simulink model "A_OnTheGo_PID"  (R2026a)
settings: Solver=daessc  StopTime=10
undefined symbols (not defined in the file): motor, RotateMass, X, Y, Z
libraries: sm_lib x823, nesl_utility x31, simulink x1
(part 1 of 25)
settings Model: Creator=fdors  LastModifiedBy=ctalle16
settings SimscapeCC: SimscapeNominalValues="[{\"value\":\"1\",\"unit\":\"A\"},{\"value\":\"1\",\"unit\":\"bar\"},{\"value\":\"1\",\"unit\":\"cm^2\"},{\"value\":\"1\",\"unit\":\"cm^3/s\"},{\"value\":\"1\",\"unit\":\"kJ/kg\"},{\"value\":\"1\",\"unit\":\"kW\"},{\"value\":\"1\",\"unit\":\"l\"},{\"value\":\"1\",\"unit\":\"N\"},{\"value\":\"1\",\"unit\":\"N*m\"},{\"value\":\"1\",\"unit\":\"V\"}]"  SimscapeLogType=none  SimscapeLogDataHistory=5000.0
settings ExplorerConfigSet: InternalSimMechanicsExplorerSettings=|
  | <ExplorerConfiguration>
  | 
  |   <canonicalview>planar_xy</canonicalview>
  | 
  |   <TilePanel>
  |     <TileInfo>
  |       <Tiles Columns="1" Count="1" Height="985" Rows="1" Width="1142">
  |         <Row Weight="1"/>
  |         <Column Weight="1"/>
  |         <Tile Height="1" Width="1" X="0" Y="0"/>
  |       </Tiles>
  |     </TileInfo>
  |     <SceneInfo>
  |       <SceneViewer>
  |         <IsThisViewStd>
  |           <IsStandardView>off</IsStandardView>
  |           <StandardViewName>Front</StandardViewName>
  |         </IsThisViewStd>
  |         <BGColor>
  |           <R>1</R>
  |           <G>1</G>
  |           <B>1</B>
  |           <A>1</A>
  |         </BGColor>
  |         <Camera>
  |           <DoPerspective>off</DoPerspective>
  |           <Position>
  |             <X>0.67806105182753051</X>
  |             <Y>0.74872215079128168</Y>
  |             <Z>0.72031476009846773</Z>
  |           </Position>
  |           <Center>
  |             <X>-0.014616720378398888</X>
  |             <Y>0.056044378585352252</Y>
  |             <Z>0.027636987892538302</Z>
  |           </Center>
  |           <Up>
  |             <X>-0.40824829046386302</X>
  |             <Y>0.81649658092772603</Y>
  |             <Z>-0.40824829046386302</Z>
  |           </Up>
  |           <XLim>0.17072201332507064</XLim>
  |           <YLim>0.17072201332507064</YLim>
  |           <ViewLimDist>0.01</ViewLimDist>
  |         </Camera>
  |       </SceneViewer>
  |     </SceneInfo>
  |   </TilePanel>
  | 
  |   <MechEditorPanel>
  |     <GfxPanelCameraMap/>
  |     <Cameras/>
  |     <VideoCreator>
  |       <IncludeTiles>All</IncludeTiles>
  |       <IncludeTime>on</IncludeTime>
  |       <IncludeWorldFrame>off</IncludeWorldFrame>
  |       <PlaybackSpeedRatio>1</PlaybackSpeedRatio>
  |       <FrameRate>30</FrameRate>
  |       <FrameSize>auto</FrameSize>
  |       <VideoFormat>UncompressedAVI</VideoFormat>
  |     </VideoCreator>
  |   </MechEditorPanel>
  | 
  |   <PlaybackSettings>
  |     <PlaybackSpeedFactor>1</PlaybackSpeedFactor>
  |   </PlaybackSettings>
  | 
  | </ExplorerConfiguration>

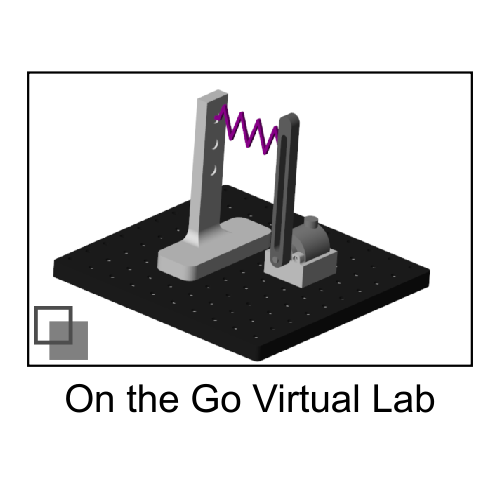
[thumbnail: Simulink's stored preview of the top-level diagram]
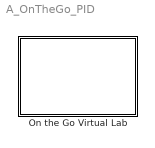
== system A_OnTheGo_PID ==
  On the Go Virtual Lab : Subsystem  Variant=on  VariantControlMode=label  VariantControl=On the Go Virtual Lab  LabelModeActiveChoice=Pendulum
      mask Display: image('upright mask cover.png');

== system A_OnTheGo_PID/On the Go Virtual Lab ==
  note: Rotating Unbalanced
  note: Pendulum
  note: X Theta
  note: Upright Pendulum
  note: Translational Rail
  note: Horizontal Pendulum
  Horizontal Pendulum : Subsystem  VariantControl=Horizontal Pendulum  mask{response_type=Forced, int_ang_dis=10, amp=0, f=0, spring1=on, s1=40, d1=.01, spring2=on, s2=40, d2=.01, spring3=on, s3=40, d3=.01, spring4=on, s4=40, d4=.01, mass=20}
      mask prompts: response_type "Response Type"; int_ang_dis "Inital Angular Displacement (deg):"; amp "Amplitude (deg):"; f "Frequency (rad/s):"; spring1 "Spring 1"; s1 "Stiffness (N/m):"; d1 "Damping [N(m/s)]:"; spring2 "Spring 2"; s2 "Stiffness (N/m):"; d2 "Damping [N(m/s)]:"; spring3 "Spring 3"; s3 "Stiffness (N/m):"; d3 "Damping [N(m/s)]:"; spring4 "Spring 4"; s4 "Stiffness (N/m):"; d4 "Damping [N(m/s)]:"; mass "Mass of Pendulum (g):"
      mask init:
      | switch response_type
      |     case 1
      |         set_param('A_OnTheGo_PID/On the Go Virtual Lab/Horizontal Pendulum/free','Commented','off')
      |         set_param('A_OnTheGo_PID/On the Go Virtual Lab/Horizontal Pendulum/forced','Commented','on')
      |     case 2
      |         set_param('A_OnTheGo_PID/On the Go Virtual Lab/Horizontal Pendulum/free','Commented','on')
      |         set_param('A_OnTheGo_PID/On the Go Virtual Lab/Horizontal Pendulum/forced','Commented','off')
      | end
      mask TypeOptions response_type: Free | Forced
      mask Callback response_type:
      | maskValues = get_param(gcb, 'MaskValues');
      | 
      | % Get the value of the first parameter (response_type)
      | response_type = maskValues{1};  % assuming it's the first parameter
      | 
      | % Set visibility based on the selected response_type
      | switch response_type
      |     case 'Free'
      |         set_param(gcb, 'MaskVisibilities', {'on', 'on', 'off', 'off', 'on','on','on','on','on','on','on','on','on','on','on','on','on'});
      |     case 'Forced'
      |         set_param(gcb, 'MaskVisibilities', {'on', 'off', 'on', 'on', 'on','on','on','on','on','on','on','on','on','on','on','on','on'});
      | end
      mask Callback spring1:
      | x=get_param(gcb,'spring1');
      | if strcmp(x,'on')
      |     set_param('A_OnTheGo_PID/On the Go Virtual Lab/Horizontal Pendulum/one','Commented','off')
      | elseif strcmp(x,'off')
      |     set_param('A_OnTheGo_PID/On the Go Virtual Lab/Horizontal Pendulum/one','Commented','on')
      | end
      mask Callback spring2:
      | x=get_param(gcb,'spring2');
      | if strcmp(x,'on')
      |     set_param('A_OnTheGo_PID/On the Go Virtual Lab/Horizontal Pendulum/two','Commented','off')
      | elseif strcmp(x,'off')
      |     set_param('A_OnTheGo_PID/On the Go Virtual Lab/Horizontal Pendulum/two','Commented','on')
      | end
      mask Callback spring3:
      | x=get_param(gcb,'spring3');
      | if strcmp(x,'on')
      |     set_param('A_OnTheGo_PID/On the Go Virtual Lab/Horizontal Pendulum/three','Commented','off')
      | elseif strcmp(x,'off')
      |     set_param('A_OnTheGo_PID/On the Go Virtual Lab/Horizontal Pendulum/three','Commented','on')
      | end
      mask Callback spring4:
      | x=get_param(gcb,'spring4');
      | if strcmp(x,'on')
      |     set_param('A_OnTheGo_PID/On the Go Virtual Lab/Horizontal Pendulum/four','Commented','off')
      | elseif strcmp(x,'off')
      |     set_param('A_OnTheGo_PID/On the Go Virtual Lab/Horizontal Pendulum/four','Commented','on')
      | end
      mask DialogControl Container2 Prompt: Response
      mask DialogControl Container3 Prompt: Free
      mask DialogControl Container4 Prompt: Forced
      mask DialogControl Container5 Prompt: Springs
      mask DialogControl Container6 Prompt: Spring 1
      mask DialogControl Container7 Prompt: Spring 2
      mask DialogControl Container8 Prompt: Spring 3
      mask DialogControl Container9 Prompt: Spring 4
      mask DialogControl Container10 Prompt: Mass
      mask Display: image('mask cover horizontal pen.png');
  Pendulum : Subsystem  VariantControl=Pendulum  mask{response_type=PID, m=10, c=.000005, disp=45, amp=.005, freq=10, pid_input=Square Wave, p=0.05, I=0, d=0.003, s=0, a=15, f=1}
      mask prompts: response_type "Response Type"; m "Tip Load Mass (g):"; c "Damping Coefficient"; disp "Initial Displacement (Deg):"; amp "Amplitude (N*m):"; freq "Frequency (rad/s):"; pid_input "Desired Response"; p "Proportional"; I "Integral"; d "Derivative"; s "Step"; a "Amplitude"; f "Frequency"
      mask init:
      | switch response_type
      |     case 1
      |         set_param('A_OnTheGo_PID/On the Go Virtual Lab/Pendulum/Free','Commented','off');
      |         set_param('A_OnTheGo_PID/On the Go Virtual Lab/Pendulum/Forced','Commented','on');
      |         set_param('A_OnTheGo_PID/On the Go Virtual Lab/Pendulum/PID','Commented','on');
      |     case 2
      |         set_param('A_OnTheGo_PID/On the Go Virtual Lab/Pendulum/Free','Commented','on');
      |         set_param('A_OnTheGo_PID/On the Go Virtual Lab/Pendulum/Forced','Commented','off');
      |         set_param('A_OnTheGo_PID/On the Go Virtual Lab/Pendulum/PID','Commented','on');
      |     case 3
      |         set_param('A_OnTheGo_PID/On the Go Virtual Lab/Pendulum/Free','Commented','on');
      |         set_param('A_OnTheGo_PID/On the Go Virtual Lab/Pendulum/Forced','Commented','on');
      |         set_param('A_OnTheGo_PID/On the Go Virtual Lab/Pendulum/PID','Commented','off');
      | end
      | switch pid_input
      |     case 1
      |         set_param('A_OnTheGo_PID/On the Go Virtual Lab/Pendulum/PID/Square','Commented','on');
      |         set_param('A_OnTheGo_PID/On the Go Virtual Lab/Pendulum/PID/Constant','Commented','off');
      |     case 2
      |         set_param('A_OnTheGo_PID/On the Go Virtual Lab/Pendulum/PID/Square','Commented','off');
      |         set_param('A_OnTheGo_PID/On the Go Virtual Lab/Pendulum/PID/Constant','Commented','on');
      | end
      mask TypeOptions response_type: Free | Forced | PID
      mask Callback response_type:
      | maskValues = get_param(gcb, 'MaskValues');
      | response_type = maskValues{1};
      | pid = maskValues{7};
      | 
      | if response_type == "Free"
      |     set_param(gcb, 'MaskVisibilities', {'on', 'on', 'on', 'on', 'off', 'off', 'off', 'off', 'off', 'off', 'off', 'off', 'off'})
      | elseif response_type == "Forced"
      |     set_param(gcb, 'MaskVisibilities', {'on', 'on', 'on', 'off', 'on', 'on', 'off', 'off', 'off', 'off', 'off', 'off', 'off'})
      | else
      |     if pid == "Constant"
      |         set_param(gcb, 'MaskVisibilities', {'on', 'on', 'on', 'off', 'off', 'off', 'on', 'on', 'on', 'on', 'on', 'off', 'off'})
      |     else
      |         set_param(gcb, 'MaskVisibilities', {'on', 'on', 'on', 'off', 'off', 'off', 'on', 'on', 'on', 'on', 'off', 'on', 'on'})
      |     end
      | end
      mask TypeOptions pid_input: Constant | Square Wave
      mask Callback pid_input:
      | maskValues = get_param(gcb, 'MaskValues');
      | pid = maskValues{7};
      | response_type = maskValues{1};
      | 
      | if response_type == "Free"
      |     set_param(gcb, 'MaskVisibilities', {'on', 'on', 'on', 'on', 'off', 'off', 'off', 'off', 'off', 'off', 'off', 'off', 'off'})
      | elseif response_type == "Forced"
      |     set_param(gcb, 'MaskVisibilities', {'on', 'on', 'on', 'off', 'on', 'on', 'off', 'off', 'off', 'off', 'off', 'off', 'off'})
      | else
      |     if pid == "Constant"
      |         set_param(gcb, 'MaskVisibilities', {'on', 'on', 'on', 'off', 'off', 'off', 'on', 'on', 'on', 'on', 'on', 'off', 'off'})
      |     else
      |         set_param(gcb, 'MaskVisibilities', {'on', 'on', 'on', 'off', 'off', 'off', 'on', 'on', 'on', 'on', 'off', 'on', 'on'})
      |     end
      | end
      mask DialogControl Free Prompt: Free
      mask DialogControl Forced Prompt: Forced
      mask DialogControl PID Prompt: PID
      mask DialogControl pid_gains Prompt: Gains
      mask DialogControl step_function Prompt: Constant
      mask DialogControl square_wave Prompt: Square Wave
      mask Display: image('Pendulum mask cover.png');
  Rotating Unbalanced : Subsystem  VariantControl=Rotating  mask{V=463, k=1, c=.1, m1=20, m2=20, m3=20, m4=0}
      mask prompts: V "Motor Speed (RPM)"; k "Spring Coefficient"; c "Friction Damping Coefficient"; m1 "Mass 1 (g)"; m2 "Mass 2 (g)"; m3 "Mass 3 (g)"; m4 "Mass 4 (g)"
      mask Callback m1:
      | maskValues = get_param(gcb, 'MaskValues');
      | if maskValues{4} == '0'
      |     set_param('A_OnTheGo_PID/On the Go Virtual Lab/Rotating Unbalanced/Mass 1','Commented','on');
      | else
      |     set_param('A_OnTheGo_PID/On the Go Virtual Lab/Rotating Unbalanced/Mass 1','Commented','off');
      | end
      mask Callback m2:
      | maskValues = get_param(gcb, 'MaskValues');
      | if maskValues{5} == '0'
      |     set_param('A_OnTheGo_PID/On the Go Virtual Lab/Rotating Unbalanced/Mass 2','Commented','on');
      | else
      |     set_param('A_OnTheGo_PID/On the Go Virtual Lab/Rotating Unbalanced/Mass 2','Commented','off');
      | end
      mask Callback m3:
      | maskValues = get_param(gcb, 'MaskValues');
      | if maskValues{6} == '0'
      |     set_param('A_OnTheGo_PID/On the Go Virtual Lab/Rotating Unbalanced/Mass 3','Commented','on');
      | else
      |     set_param('A_OnTheGo_PID/On the Go Virtual Lab/Rotating Unbalanced/Mass 3','Commented','off');
      | end
      mask Callback m4:
      | maskValues = get_param(gcb, 'MaskValues');
      | if maskValues{7} == '0'
      |     set_param('A_OnTheGo_PID/On the Go Virtual Lab/Rotating Unbalanced/Mass 4','Commented','on');
      | else
      |     set_param('A_OnTheGo_PID/On the Go Virtual Lab/Rotating Unbalanced/Mass 4','Commented','off');
      | end
      mask DialogControl ParameterGroupVar Prompt: Motor Parameters
      mask DialogControl Container3 Prompt: Vibration Parameters
      mask DialogControl Container4 Prompt: Mass Parameters
      mask Display: image('Rotating Unbalanced.png');
  Translational Rail : Subsystem  VariantControl=Translational Rail  mask{spr_k=600, spr_d=1, rail_d=.35, mass1=50, mass_c=20, response_type=Forced, int_disp=3.2, amp=0, f=0}
      mask prompts: spr_k "Spring Stiffness (N/m):"; spr_d "Spring Damping Coefficient [N/(m/s]:"; rail_d "Rail Fricition Coefficient [N/(m/s)]:"; mass1 "Mass on cart (g):"; mass_c "Cart Mass (g):"; response_type "Response Type:"; int_disp "Intial Displacement (cm):"; amp "Amplitude (cm):"; f "Frequency (rad/s):"
      mask init:
      | switch response_type
      |     case 1
      |         set_param('A_OnTheGo_PID/On the Go Virtual Lab/Translational Rail/free','Commented','off')
      |         set_param('A_OnTheGo_PID/On the Go Virtual Lab/Translational Rail/forced','Commented','on')
      |     case 2
      |         set_param('A_OnTheGo_PID/On the Go Virtual Lab/Translational Rail/free','Commented','on')
      |         set_param('A_OnTheGo_PID/On the Go Virtual Lab/Translational Rail/forced','Commented','off')
      | end
      mask TypeOptions response_type: Free | Forced
      mask Callback response_type:
      | maskValues = get_param(gcb, 'MaskValues');
      | 
      | % Get the value of the first parameter (response_type)
      | response_type = maskValues{6};  % assuming it's the first parameter
      | 
      | % Set visibility based on the selected response_type
      | switch response_type
      |     case 'Free'
      |         set_param(gcb, 'MaskVisibilities', {'on', 'on','on','on','on','on','on','off','off'});
      |     case 'Forced'
      |         set_param(gcb, 'MaskVisibilities', {'on', 'on', 'on', 'on','on','on','off','on','on'});
      | end
      mask DialogControl ParameterGroupVar Prompt: System Parameters
      mask DialogControl Container3 Prompt: Response
      mask DialogControl free Prompt: Free
      mask DialogControl forced Prompt: Forced
      mask Display: image('translational mask image.png');
  Upright Pendulum : Subsystem  VariantControl=Upright Pendulum  mask{response_type=PID, ang_dis=2.5, amp=0, fr=0, pid_input=Square Wave, p=0.075, I=0.025, d=0.005, s=0, a=10, f=1, spring_top=on, k_top=70, d_top=.35, spring_middle=off, k_middle=70, d_middle=.35, spring_bottom=on, k_bottom=70, d_bottom=.35}
      mask prompts: response_type "Response type:"; ang_dis "Initial Angular Displacement (deg):"; amp "Amplitude"; fr "Frequency (rad/sec):"; pid_input "Desired Input"; p "Proportional"; I "Integral"; d "Derivative"; s "Constant"; a "Amplitude"; f "Frequency"; spring_top "Top"; k_top "Spring Stiffness (N/m):"; d_top "Spring Damping [N/(m/s)]:"; spring_middle "Middle"; k_middle "Spring Stiffness (N/m):"; d_middle "Spring Damping [N/(m/s)]:"; spring_bottom "Bottom"; k_bottom "Spring Stiffness (N/m):"; d_bottom "Spring Damping [N/(m/s)]:"
      mask init:
      | switch response_type
      |     case 1
      |         set_param('A_OnTheGo_PID/On the Go Virtual Lab/Upright Pendulum/free','Commented','off');
      |         set_param('A_OnTheGo_PID/On the Go Virtual Lab/Upright Pendulum/forced','Commented','on');
      |         set_param('A_OnTheGo_PID/On the Go Virtual Lab/Upright Pendulum/PID','Commented','on');
      |     case 2
      |         set_param('A_OnTheGo_PID/On the Go Virtual Lab/Upright Pendulum/free','Commented','on');
      |         set_param('A_OnTheGo_PID/On the Go Virtual Lab/Upright Pendulum/forced','Commented','off');
      |         set_param('A_OnTheGo_PID/On the Go Virtual Lab/Upright Pendulum/PID','Commented','on');
      |     case 3
      |         set_param('A_OnTheGo_PID/On the Go Virtual Lab/Upright Pendulum/free','Commented','on');
      |         set_param('A_OnTheGo_PID/On the Go Virtual Lab/Upright Pendulum/forced','Commented','on');
      |         set_param('A_OnTheGo_PID/On the Go Virtual Lab/Upright Pendulum/PID','Commented','off');
      | end
      | 
      | switch pid_input
      |     case 1
      |         set_param('A_OnTheGo_PID/On the Go Virtual Lab/Upright Pendulum/PID/Constant','Commented','off');
      |         set_param('A_OnTheGo_PID/On the Go Virtual Lab/Upright Pendulum/PID/Square','Commented','on');
      |     case 2
      |         set_param('A_OnTheGo_PID/On the Go Virtual Lab/Upright Pendulum/PID/Constant','Commented','on');
      |         set_param('A_OnTheGo_PID/On the Go Virtual Lab/Upright Pendulum/PID/Square','Commented','off');
      | end
      mask TypeOptions response_type: Free | Forced | PID
      mask Callback response_type:
      | maskValues = get_param(gcb, 'MaskValues');
      | 
      | % Get the value of the first parameter (response_type)
      | response_type = maskValues{1};  % assuming it's the first parameter
      | 
      | % Set visibility based on the selected response_type
      | switch response_type
      |     case 'Free'
      |         set_param(gcb, 'MaskVisibilities', {'on', 'on', 'off', 'off', 'off', 'off', 'off', 'off', 'off', 'off', 'off', 'on','on','on','on','on','on','on','on','on'});
      |     case 'Forced'
      |         set_param(gcb, 'MaskVisibilities', {'on', 'off', 'on', 'on', 'off', 'off', 'off', 'off', 'off', 'off', 'off', 'on','on','on','on','on','on','on','on','on'});
      |     case 'PID'
      |         set_param(gcb, 'MaskVisibilities', {'on', 'off', 'off', 'off', 'on', 'on', 'on', 'on', 'on', 'on', 'on', 'on','on','on','on','on','on','on','on','on'});
      | end
      mask TypeOptions pid_input: Constant | Square Wave
      mask Callback spring_top:
      | x=get_param(gcb,'spring_top');
      | if strcmp(x,'on')
      |     set_param('A_OnTheGo_PID/On the Go Virtual Lab/Upright Pendulum/top','Commented','off');
      | elseif strcmp(x,'off')
      |     set_param('A_OnTheGo_PID/On the Go Virtual Lab/Upright Pendulum/top','Commented','on');
      | end
      mask Callback spring_middle:
      | x=get_param(gcb,'spring_middle');
      | if strcmp(x,'on')
      |     set_param('A_OnTheGo_PID/On the Go Virtual Lab/Upright Pendulum/middle','Commented','off');
      | elseif strcmp(x,'off')
      |     set_param('A_OnTheGo_PID/On the Go Virtual Lab/Upright Pendulum/middle','Commented','on');
      | end
      mask Callback spring_bottom:
      | x=get_param(gcb,'spring_bottom');
      | if strcmp(x,'on')
      |     set_param('A_OnTheGo_PID/On the Go Virtual Lab/Upright Pendulum/bottom','Commented','off');
      | elseif strcmp(x,'off')
      |     set_param('A_OnTheGo_PID/On the Go Virtual Lab/Upright Pendulum/bottom','Commented','on');
      | end
      mask DialogControl Container4 Prompt: Response
      mask DialogControl Container1 Prompt: Free
      mask DialogControl Container6 Prompt: Forced
      mask DialogControl Container11 Prompt: PID
      mask DialogControl Container12 Prompt: Gains
      mask DialogControl Container13 Prompt: Constant
      mask DialogControl Container14 Prompt: Square Wave
      mask DialogControl Container5 Prompt: Spring
      mask DialogControl Container7 Prompt: Spring Location
      mask DialogControl Container8 Prompt: Top
      mask DialogControl Container9 Prompt: Middle
      mask DialogControl Container10 Prompt: Bottom
      mask Display: image('upright mask cover.png');
  X Theta : Subsystem  VariantControl=X Theta  mask{response_type=Free, ang_dis=0, amp=30, f=1, initial_dis=2.500, rail_c=.1, cart_mass=10, spring_left=on, spring_l_k=20, spring_l_d=.1, spring_right=off, spring_r_k=20, spring_r_d=.1}
      mask prompts: response_type "Response Type:"; ang_dis "Initial Angular Displacement (deg):"; amp "Amplitude (deg):"; f "Frequency (rad/s):"; initial_dis "Initial Cart Displacement (cm):"; rail_c "Rail Damping [N(m/s)]:"; cart_mass "Mass of Cart (g):"; spring_left "Left"; spring_l_k "Stiffness (N/m):"; spring_l_d "Damping [(N/(m/s)]:"; spring_right "Right"; spring_r_k "Stiffness (N/m):"; spring_r_d "Damping [(N/(m/s)]:"
      mask init:
      | switch response_type
      |     case 1
      |         set_param('A_OnTheGo_PID/On the Go Virtual Lab/X Theta/Free','Commented','off');
      |         set_param('A_OnTheGo_PID/On the Go Virtual Lab/X Theta/Forced','Commented','on');
      |     case 2
      |         set_param('A_OnTheGo_PID/On the Go Virtual Lab/X Theta/Free','Commented','on');
      |         set_param('A_OnTheGo_PID/On the Go Virtual Lab/X Theta/Forced','Commented','off');  
      | end
      mask TypeOptions response_type: Free | Forced
      mask Callback response_type:
      | maskValues = get_param(gcb, 'MaskValues');
      | response_type = maskValues{1};  % response_type is first in list
      | 
      | % Get existing visibilities
      | vis = get_param(gcb, 'MaskVisibilities');
      | 
      | % Start with all visible
      | newVis = {'on', 'on', 'on', 'on', 'on', 'on', 'on', 'on', 'on', 'on', 'on', 'on', 'on'};
      | 
      | switch response_type
      |     case 'Free'
      |         newVis{3} = 'off';  % amp
      |         newVis{4} = 'off';  % f
      |         newVis{2} = 'on';
      |     case 'Forced'
      |         newVis{3} = 'on';   % amp
      |         newVis{4} = 'on';   % f
      |         newVis{2} = 'off';
      | end
      | 
      | set_param(gcb, 'MaskVisibilities', newVis);
      mask Callback spring_left:
      | x=get_param(gcb,'spring_left');
      | if strcmp(x,'on')
      |     set_param('A_OnTheGo_PID/On the Go Virtual Lab/X Theta/left','Commented','off');
      | elseif strcmp(x,'off')
      |     set_param('A_OnTheGo_PID/On the Go Virtual Lab/X Theta/left','Commented','on');
      | end
      mask Callback spring_right:
      | x=get_param(gcb,'spring_right');
      | if strcmp(x,'on')
      |     set_param('A_OnTheGo_PID/On the Go Virtual Lab/X Theta/right','Commented','off');
      | elseif strcmp(x,'off')
      |     set_param('A_OnTheGo_PID/On the Go Virtual Lab/X Theta/right','Commented','on');
      | end
      mask DialogControl Container6 Prompt: Response
      mask DialogControl Container7 Prompt: Free
      mask DialogControl Container8 Prompt: Forced
      mask DialogControl Container5 Prompt: System Parameters
      mask DialogControl Container2 Prompt: Springs
      mask DialogControl Container3 Prompt: Left Spring
      mask DialogControl Container4 Prompt: Right Spring
      mask Display: image('xTheta mask image.png');

== system A_OnTheGo_PID/On the Go Virtual Lab/Horizontal Pendulum ==
  Mechanism Configuration : sm_lib/Utilities/Mechanism Configuration  UniformGravity=None  GravityVector=[0 0 -9.80665]  GravityVectorUnits=m/s^2  LinearizationDelta=0.001  JointModeTransitionNonlinearIterations=2
  Rigid Transform1 : sm_lib/Frames and Transforms/Rigid Transform  RotationMethod=None  FollAlignAxisA=+X  BaseAlignAxisA=+Y  FollAlignAxisB=+Y  BaseAlignAxisB=+Z  RotationStandardAxis=+Z  RotationAngle=0  RotationAngleUnits=deg  RotationArbitraryAxis=[0 0 1]  RotationSequenceAxes=FollowerAxes  RotationSequence=XYX  RotationSequenceAngles=[0 0 0]  RotationSequenceAnglesUnits=deg  RotationMatrix=[1 0 0;0 1 0;0 0 1]  Quaternion=[1 0 0 0]  TranslationMethod=Cartesian  TranslationCartesianOffset=[136.484e-6 -1.75e-3 0]  TranslationCartesianOffsetUnits=m  TranslationStandardAxis=+Z  TranslationStandardOffset=0  TranslationStandardOffsetUnits=m  TranslationROffset=0  TranslationROffsetUnits=m  TranslationThetaOffset=0  TranslationThetaOffsetUnits=deg  TranslationZOffset=0  TranslationZOffsetUnits=m
  Rigid Transform2 : sm_lib/Frames and Transforms/Rigid Transform  RotationMethod=None  FollAlignAxisA=+X  BaseAlignAxisA=+Y  FollAlignAxisB=+Y  BaseAlignAxisB=+Z  RotationStandardAxis=+Z  RotationAngle=0  RotationAngleUnits=deg  RotationArbitraryAxis=[0 0 1]  RotationSequenceAxes=FollowerAxes  RotationSequence=XYX  RotationSequenceAngles=[0 0 0]  RotationSequenceAnglesUnits=deg  RotationMatrix=[1 0 0;0 1 0;0 0 1]  Quaternion=[1 0 0 0]  TranslationMethod=Cartesian  TranslationCartesianOffset=[136.484e-6 -1.75e-3 0]  TranslationCartesianOffsetUnits=m  TranslationStandardAxis=+Z  TranslationStandardOffset=0  TranslationStandardOffsetUnits=m  TranslationROffset=0  TranslationROffsetUnits=m  TranslationThetaOffset=0  TranslationThetaOffsetUnits=deg  TranslationZOffset=0  TranslationZOffsetUnits=m
  Rigid Transform3 : sm_lib/Frames and Transforms/Rigid Transform  RotationMethod=None  FollAlignAxisA=+X  BaseAlignAxisA=+Y  FollAlignAxisB=+Y  BaseAlignAxisB=+Z  RotationStandardAxis=+Z  RotationAngle=0  RotationAngleUnits=deg  RotationArbitraryAxis=[0 0 1]  RotationSequenceAxes=FollowerAxes  RotationSequence=XYX  RotationSequenceAngles=[0 0 0]  RotationSequenceAnglesUnits=deg  RotationMatrix=[1 0 0;0 1 0;0 0 1]  Quaternion=[1 0 0 0]  TranslationMethod=Cartesian  TranslationCartesianOffset=[-163.501e-6 -1.75e-3 0]  TranslationCartesianOffsetUnits=m  TranslationStandardAxis=+Z  TranslationStandardOffset=0  TranslationStandardOffsetUnits=m  TranslationROffset=0  TranslationROffsetUnits=m  TranslationThetaOffset=0  TranslationThetaOffsetUnits=deg  TranslationZOffset=0  TranslationZOffsetUnits=m
  Rigid Transform4 : sm_lib/Frames and Transforms/Rigid Transform  RotationMethod=None  FollAlignAxisA=+X  BaseAlignAxisA=+Y  FollAlignAxisB=+Y  BaseAlignAxisB=+Z  RotationStandardAxis=+Z  RotationAngle=0  RotationAngleUnits=deg  RotationArbitraryAxis=[0 0 1]  RotationSequenceAxes=FollowerAxes  RotationSequence=XYX  RotationSequenceAngles=[0 0 0]  RotationSequenceAnglesUnits=deg  RotationMatrix=[1 0 0;0 1 0;0 0 1]  Quaternion=[1 0 0 0]  TranslationMethod=Cartesian  TranslationCartesianOffset=[-163.501e-6 -1.75e-3 0]  TranslationCartesianOffsetUnits=m  TranslationStandardAxis=+Z  TranslationStandardOffset=0  TranslationStandardOffsetUnits=m  TranslationROffset=0  TranslationROffsetUnits=m  TranslationThetaOffset=0  TranslationThetaOffsetUnits=deg  TranslationZOffset=0  TranslationZOffsetUnits=m
  Solver Configuration : nesl_utility/Solver Configuration  PhysicalDomain=network_engine_domain  SubClassName=solver  LeftPortType=input  RightPortType=generic  Tones=[]  Harmonics=[]  SimulateNoise=off  Profile=off  UseLocalSampling=off  EnableSwitchedLinearOptims=on  FrequencyDomain=off  UseCCode=off  RelTol=0.001  AbsTol=0.001  MinStep=1e-09  ToWorkspace=off  RevertToSquareIcSolve=off  NumHomotopyIterations=100  PhasorMode=off  PhasorModeNumHarmonics=1  ConsistencySolver=NEWTON_XTOL_AFTER_FTOL  CanonicalOrdering=UNORDERED  OptimizeIntermediates=UNOPTIMIZED  IndexReductionMethod=DerivativeReplacement  DoDC=off  ResidualTolerance=1e-09  ConsistencyTolSource=GLOBAL  ConsistencyAbsTol=0.001  ConsistencyRelTol=0.001  ConsistencyTolFactor=0.001  UseLocalSolver=off  LocalSolverChoice=NE_BACKWARD_EULER_ADVANCER  ResolveIndetEquations=on  FunctionEvalNumThread=1  LocalSolverSampleTime=0.001  DoFixedCost=off  MaxNonlinIter=3  MaxModeIter=2  ComputeImpulses=off  ImpulseIterations=2  LinearAlgebra=auto  LinearAlgebraNumThread=0  EquationFormulation=NE_TIME_EF  DelaysMemoryBudget=1024  AutomaticFiltering=on  FilteringTimeConstant=0.001  PartitionStorageMethod=AS_NEEDED  PartitionMemoryBudget=1024  PartitionMethod=ROBUST  MultibodyUseLocalSolver=off  MultibodyLocalSolverChoice=ODE1  MultibodyLocalSolverSampleTime=0.001
  Weld Joint{,1..3} (4 alike) : sm_lib/Joints/Weld Joint  JointMode=Normal  CompositeWrenchDir=FollowerOnBase  CompositeWrenchFrame=BaseFrame  SenseConstraintForce=off  SenseConstraintTorque=off  SenseTotalForce=off  SenseTotalTorque=off
  World Frame : sm_lib/Frames and Transforms/World Frame
  encoder : sm_lib/Body Elements/File Solid  ExtGeomFileName=taiss encoder.STEP  UnitType=FromFile  ExtGeomFileUnits=m  StepReaderType=HEX  ExportConvexHullGeometry=off  InertiaType=CalculateFromGeometry  BasedOnType=Mass  Density=1000  DensityUnits=kg/m^3  Mass=1  MassUnits=kg  CenterOfMass=[0 0 0]  CenterOfMassUnits=m  MomentsOfInertia=[1 1 1]  MomentsOfInertiaUnits=kg*m^2  ProductsOfInertia=[0 0 0]  ProductsOfInertiaUnits=kg*m^2  GraphicType=FromGeometry  MarkerShape=Sphere  MarkerSize=10  GraphicVisPropType=SimpleVisualProperties  GraphicDiffuseColor=[0.9412 0.9412 0.9412]  GraphicOpacity=1  GraphicSpecularColor=[0.5 0.5 0.5 1.0]  GraphicAmbientColor=[0.15 0.15 0.15 1.0]  GraphicEmissiveColor=[0.0 0.0 0.0 1.0]  GraphicShininess=75  DoExposeReferenceFrame=off  SerializedFrames=<Frames><Frame><Id>Frame1</Id><Value><Name>F1</Name><Origin><Source>GeometricFeature</Source><FeatureName>planar surface 2</FeatureName></Origin><PrimaryAxis><DefinedDirection>+Z</DefinedDirection><Source>ReferenceFrame</Source><SourceDirection>+Y</SourceDirection><FeatureName></FeatureName></PrimaryAxis><SecondaryAxis><DefinedDirection>+X</DefinedDirection><Source>ReferenceFrame</Source><SourceDirection>-X</SourceDirection><FeatureName></FeatureName></SecondaryAxis></Value></Frame><Frame><Id>Frame2</Id><Value><Name>F2</Name><Origin><Source>GeometricFeature</Source><FeatureName>circular curve 4</FeatureName></Origin><PrimaryAxis><DefinedDirection>+Z</DefinedDirection><Source>ReferenceFrame</Source><SourceDirection>+Z</SourceDirection><FeatureName></FeatureName></PrimaryAxis><SecondaryAxis><DefinedDirection>+X</DefinedDirection><Source>ReferenceFrame</Source><SourceDirection>+X</SourceDirection><FeatureName></FeatureName></SecondaryAxis></Value></Frame></Frames>
  encoder holder : sm_lib/Body Elements/File Solid  ExtGeomFileName=Encoder Holder Horizontal pend.STEP  UnitType=FromFile  ExtGeomFileUnits=m  StepReaderType=HEX  ExportConvexHullGeometry=off  InertiaType=CalculateFromGeometry  BasedOnType=Mass  Density=1000  DensityUnits=kg/m^3  Mass=1  MassUnits=kg  CenterOfMass=[0 0 0]  CenterOfMassUnits=m  MomentsOfInertia=[1 1 1]  MomentsOfInertiaUnits=kg*m^2  ProductsOfInertia=[0 0 0]  ProductsOfInertiaUnits=kg*m^2  GraphicType=FromGeometry  MarkerShape=Sphere  MarkerSize=10  GraphicVisPropType=SimpleVisualProperties  GraphicDiffuseColor=[0.5 0.5 0.5]  GraphicOpacity=1  GraphicSpecularColor=[0.5 0.5 0.5 1.0]  GraphicAmbientColor=[0.15 0.15 0.15 1.0]  GraphicEmissiveColor=[0.0 0.0 0.0 1.0]  GraphicShininess=75  DoExposeReferenceFrame=off  SerializedFrames=<Frames><Frame><Id>Frame1</Id><Value><Name>F1</Name><Origin><Source>GeometricFeature</Source><FeatureName>circular curve 6</FeatureName></Origin><PrimaryAxis><DefinedDirection>+Z</DefinedDirection><Source>ReferenceFrame</Source><SourceDirection>+Z</SourceDirection><FeatureName></FeatureName></PrimaryAxis><SecondaryAxis><DefinedDirection>+X</DefinedDirection><Source>ReferenceFrame</Source><SourceDirection>-X</SourceDirection><FeatureName></FeatureName></SecondaryAxis></Value></Frame><Frame><Id>Frame2</Id><Value><Name>F2</Name><Origin><Source>GeometricFeature</Source><FeatureName>planar surface 3</FeatureName></Origin><PrimaryAxis><DefinedDirection>+Z</DefinedDirection><Source>ReferenceFrame</Source><SourceDirection>+Z</SourceDirection><FeatureName></FeatureName></PrimaryAxis><SecondaryAxis><DefinedDirection>+X</DefinedDirection><Source>ReferenceFrame</Source><SourceDirection>+X</SourceDirection><FeatureName></FeatureName></SecondaryAxis></Value></Frame></Frames>
  forced : Subsystem
  four : Subsystem  mask{spr_k=600, spr_d=1, spr_l=71.355e-3, popup_set_z0=off, z0=0, spr_od=.02, seg_w=.003, spr_m=1e-4, spr_clr=[1 1 1], spr_opc=1}
      mask prompts: spr_k "Stiffness (N/m)"; spr_d "Damping (N/m)"; spr_l "Free Length (m)"; popup_set_z0 "Specify Initial Length"; z0 "Initial Length (m)"; spr_od "Outer Diameter (m)"; seg_w "Wire Diameter (m)"; spr_m "Total Mass (kg)"; spr_clr "Color [RGB]"; spr_opc "Opacity (0-1)"
      mask init:
      | % Number of segment used to visualize spring
      | % Fixed parameter for this block
      | spr_nseg = 7;
      | 
      | % Stems are 10% of spring length
      | coil_len = spr_l*0.9;
      | 
      | % Coil diameter is outer diameter - wire diameter
      | coil_d   = spr_od-seg_w;
      | 
      | % Determine angle between segments
      | seg_angle = atan((coil_len/spr_nseg)/coil_d)*2;
      | 
      | % Determine segment length
      | seg_l = coil_d/cos(seg_angle/2);
      | 
      | % Create profile data for segment ends
      | seg_cap_ptsA = linspace(-pi/2,pi/2,15)';
      | seg_cap_ptsB = linspace(pi/2,3*pi/2,15)';
      | extr_seg_capA = seg_w/2*[cos(seg_cap_ptsA) sin(seg_cap_ptsA)];
      | extr_seg_capB = seg_w/2*[cos(seg_cap_ptsB) sin(seg_cap_ptsB)];
      | 
      | % Create extrusion profiles for full and half segments
      | extr_seg = [...
      |     extr_seg_capA+[seg_l/2 0]
      |     extr_seg_capB-[seg_l/2 0]];
      | 
      | extr_seg_half = [...
      |     extr_seg_capA+[seg_l/4 0]
      |     extr_seg_capB-[seg_l/4 0]];
      | 
      | % Set initial length if desired
      | set_param([gcb '/Prismatic Joint1'],...
      |     'PositionTargetSpecify',get_param(gcb,('popup_set_z0')));
      mask Callback popup_set_z0:
      | maskObj = Simulink.Mask.get(gcb);
      | z0_h = maskObj.getParameter('z0');
      | z0_h.Visible = get_param(gcb,'popup_set_z0');
      | 
      | clear maskObj z0_h
  free : Subsystem  Commented=on
  one : Subsystem  mask{spr_k=600, spr_d=1, spr_l=72.496e-3, popup_set_z0=off, z0=0, spr_od=.02, seg_w=.003, spr_m=1e-4, spr_clr=[0 0 .75], spr_opc=1}
      mask prompts: spr_k "Stiffness (N/m)"; spr_d "Damping (N/m)"; spr_l "Free Length (m)"; popup_set_z0 "Specify Initial Length"; z0 "Initial Length (m)"; spr_od "Outer Diameter (m)"; seg_w "Wire Diameter (m)"; spr_m "Total Mass (kg)"; spr_clr "Color [RGB]"; spr_opc "Opacity (0-1)"
      mask init: same as A_OnTheGo_PID/On the Go Virtual Lab/Horizontal Pendulum/four
      mask Callback popup_set_z0:
      | maskObj = Simulink.Mask.get(gcb);
      | z0_h = maskObj.getParameter('z0');
      | z0_h.Visible = get_param(gcb,'popup_set_z0');
      | 
      | clear maskObj z0_h
  peg board : sm_lib/Body Elements/File Solid  ExtGeomFileName=pegboard.STEP  UnitType=FromFile  ExtGeomFileUnits=m  StepReaderType=HEX  ExportConvexHullGeometry=off  InertiaType=CalculateFromGeometry  BasedOnType=Mass  Density=1000  DensityUnits=kg/m^3  Mass=1  MassUnits=kg  CenterOfMass=[0 0 0]  CenterOfMassUnits=m  MomentsOfInertia=[1 1 1]  MomentsOfInertiaUnits=kg*m^2  ProductsOfInertia=[0 0 0]  ProductsOfInertiaUnits=kg*m^2  GraphicType=FromGeometry  MarkerShape=Sphere  MarkerSize=10  GraphicVisPropType=SimpleVisualProperties  GraphicDiffuseColor=[0.149 0.149 0.149]  GraphicOpacity=1  GraphicSpecularColor=[0.5 0.5 0.5 1.0]  GraphicAmbientColor=[0.15 0.15 0.15 1.0]  GraphicEmissiveColor=[0.0 0.0 0.0 1.0]  GraphicShininess=75  DoExposeReferenceFrame=on  SerializedFrames=<Frames><Frame><Id>Frame1</Id><Value><Name>F1</Name><Origin><Source>GeometricFeature</Source><FeatureName>circular curve 235</FeatureName></Origin><PrimaryAxis><DefinedDirection>+Z</DefinedDirection><Source>ReferenceFrame</Source><SourceDirection>+Z</SourceDirection><FeatureName></FeatureName></PrimaryAxis><SecondaryAxis><DefinedDirection>+X</DefinedDirection><Source>ReferenceFrame</Source><SourceDirection>+X</SourceDirection><FeatureName></FeatureName></SecondaryAxis></Value></Frame><Frame><Id>Frame2</Id><Value><Name>F2</Name><Origin><Source>GeometricFeature</Source><FeatureName>circular curve 267</FeatureName></Origin><PrimaryAxis><DefinedDirection>+Z</DefinedDirection><Source>ReferenceFrame</Source><SourceDirection>+Z</SourceDirection><FeatureName></FeatureName></PrimaryAxis><SecondaryAxis><DefinedDirection>+X</DefinedDirection><Source>ReferenceFrame</Source><SourceDirection>+X</SourceDirection><FeatureName></FeatureName></SecondaryAxis></Value></Frame><Frame><Id>Frame3</Id><Value><Name>F3</Name><Origin><Source>GeometricFeature</Source><FeatureName>circular curve 26</FeatureName></Origin><PrimaryAxis><DefinedDirection>+Z</DefinedDirection><Source>ReferenceFrame</Source><SourceDirection>+Z</SourceDirection><FeatureName></FeatureName></PrimaryAxis><SecondaryAxis><DefinedDirection>+X</DefinedDirection><Source>ReferenceFrame</Source><SourceDirection>+X</SourceDirection><FeatureName></FeatureName></SecondaryAxis></Value></Frame></Frames>
  pendulum arm : sm_lib/Body Elements/File Solid  ExtGeomFileName=Pendulum Project 6.STEP  UnitType=FromFile  ExtGeomFileUnits=m  StepReaderType=HEX  ExportConvexHullGeometry=off  InertiaType=CalculateFromGeometry  BasedOnType=Mass  Density=1000  DensityUnits=kg/m^3  Mass=mass  MassUnits=g  CenterOfMass=[0 0 0]  CenterOfMassUnits=m  MomentsOfInertia=[1 1 1]  MomentsOfInertiaUnits=kg*m^2  ProductsOfInertia=[0 0 0]  ProductsOfInertiaUnits=kg*m^2  GraphicType=FromGeometry  MarkerShape=Sphere  MarkerSize=10  GraphicVisPropType=SimpleVisualProperties  GraphicDiffuseColor=[0.5 0.5 0.5]  GraphicOpacity=1  GraphicSpecularColor=[0.5 0.5 0.5 1.0]  GraphicAmbientColor=[0.15 0.15 0.15 1.0]  GraphicEmissiveColor=[0.0 0.0 0.0 1.0]  GraphicShininess=75  DoExposeReferenceFrame=off  SerializedFrames=<Frames><Frame><Id>Frame1</Id><Value><Name>F1</Name><Origin><Source>GeometricFeature</Source><FeatureName>circular curve 16</FeatureName></Origin><PrimaryAxis><DefinedDirection>+Z</DefinedDirection><Source>ReferenceFrame</Source><SourceDirection>-Z</SourceDirection><FeatureName></FeatureName></PrimaryAxis><SecondaryAxis><DefinedDirection>+X</DefinedDirection><Source>ReferenceFrame</Source><SourceDirection>+X</SourceDirection><FeatureName></FeatureName></SecondaryAxis></Value></Frame><Frame><Id>Frame2</Id><Value><Name>one</Name><Origin><Source>GeometricFeature</Source><FeatureName>planar surface 12</FeatureName></Origin><PrimaryAxis><DefinedDirection>+Z</DefinedDirection><Source>ReferenceFrame</Source><SourceDirection>+Y</SourceDirection><FeatureName></FeatureName></PrimaryAxis><SecondaryAxis><DefinedDirection>+X</DefinedDirection><Source>ReferenceFrame</Source><SourceDirection>-X</SourceDirection><FeatureName></FeatureName></SecondaryAxis></Value></Frame><Frame><Id>Frame3</Id><Value><Name>two</Name><Origin><Source>GeometricFeature</Source><FeatureName>planar surface 13</FeatureName></Origin><PrimaryAxis><DefinedDirection>+Z</DefinedDirection><Source>ReferenceFrame</Source><SourceDirection>+Y</SourceDirection><FeatureName></FeatureName></PrimaryAxis><SecondaryAxis><DefinedDirection>+X</DefinedDirection><Source>ReferenceFrame</Source><SourceDirection>-X</SourceDirection><FeatureName></FeatureName></SecondaryAxis></Value></Frame><Frame><Id>Frame4</Id><Value><Name>three</Name><Origin><Source>GeometricFeature</Source><FeatureName>planar surface 11</FeatureName></Origin><PrimaryAxis><DefinedDirection>+Z</DefinedDirection><Source>ReferenceFrame</Source><SourceDirection>+Y</SourceDirection><FeatureName></FeatureName></PrimaryAxis><SecondaryAxis><DefinedDirection>+X</DefinedDirection><Source>ReferenceFrame</Source><SourceDirection>-X</SourceDirection><FeatureName></FeatureName></SecondaryAxis></Value></Frame><Frame><Id>Frame5</Id><Value><Name>four</Name><Origin><Source>GeometricFeature</Source><FeatureName>planar surface 10</FeatureName></Origin><PrimaryAxis><DefinedDirection>+Z</DefinedDirection><Source>ReferenceFrame</Source><SourceDirection>+Y</SourceDirection><FeatureName></FeatureName></PrimaryAxis><SecondaryAxis><DefinedDirection>+X</DefinedDirection><Source>ReferenceFrame</Source><SourceDirection>-X</SourceDirection><FeatureName></FeatureName></SecondaryAxis></Value></Frame></Frames>
  three : Subsystem  mask{spr_k=600, spr_d=1, spr_l=71.355e-3, popup_set_z0=off, z0=0, spr_od=.02, seg_w=.003, spr_m=1e-4, spr_clr=[1 1 1], spr_opc=1}
      mask prompts: spr_k "Stiffness (N/m)"; spr_d "Damping (N/m)"; spr_l "Free Length (m)"; popup_set_z0 "Specify Initial Length"; z0 "Initial Length (m)"; spr_od "Outer Diameter (m)"; seg_w "Wire Diameter (m)"; spr_m "Total Mass (kg)"; spr_clr "Color [RGB]"; spr_opc "Opacity (0-1)"
      mask init: same as A_OnTheGo_PID/On the Go Virtual Lab/Horizontal Pendulum/four
      mask Callback popup_set_z0:
      | maskObj = Simulink.Mask.get(gcb);
      | z0_h = maskObj.getParameter('z0');
      | z0_h.Visible = get_param(gcb,'popup_set_z0');
      | 
      | clear maskObj z0_h
  two : Subsystem  mask{spr_k=600, spr_d=1, spr_l=72.496e-3, popup_set_z0=off, z0=0, spr_od=.02, seg_w=.003, spr_m=1e-4, spr_clr=[1 1 1], spr_opc=1}
      mask prompts: spr_k "Stiffness (N/m)"; spr_d "Damping (N/m)"; spr_l "Free Length (m)"; popup_set_z0 "Specify Initial Length"; z0 "Initial Length (m)"; spr_od "Outer Diameter (m)"; seg_w "Wire Diameter (m)"; spr_m "Total Mass (kg)"; spr_clr "Color [RGB]"; spr_opc "Opacity (0-1)"
      mask init: same as A_OnTheGo_PID/On the Go Virtual Lab/Horizontal Pendulum/four
      mask Callback popup_set_z0:
      | maskObj = Simulink.Mask.get(gcb);
      | z0_h = maskObj.getParameter('z0');
      | z0_h.Visible = get_param(gcb,'popup_set_z0');
      | 
      | clear maskObj z0_h
  wall bottom : sm_lib/Body Elements/File Solid  ExtGeomFileName=Wall Project 2.STEP  UnitType=FromFile  ExtGeomFileUnits=m  StepReaderType=HEX  ExportConvexHullGeometry=off  InertiaType=CalculateFromGeometry  BasedOnType=Mass  Density=1000  DensityUnits=kg/m^3  Mass=1  MassUnits=kg  CenterOfMass=[0 0 0]  CenterOfMassUnits=m  MomentsOfInertia=[1 1 1]  MomentsOfInertiaUnits=kg*m^2  ProductsOfInertia=[0 0 0]  ProductsOfInertiaUnits=kg*m^2  GraphicType=FromGeometry  MarkerShape=Sphere  MarkerSize=10  GraphicVisPropType=SimpleVisualProperties  GraphicDiffuseColor=[0.5 0.5 0.5]  GraphicOpacity=1  GraphicSpecularColor=[0.5 0.5 0.5 1.0]  GraphicAmbientColor=[0.15 0.15 0.15 1.0]  GraphicEmissiveColor=[0.0 0.0 0.0 1.0]  GraphicShininess=75  DoExposeReferenceFrame=off  SerializedFrames=<Frames><Frame><Id>Frame1</Id><Value><Name>F1</Name><Origin><Source>GeometricFeature</Source><FeatureName>circular curve 8</FeatureName></Origin><PrimaryAxis><DefinedDirection>+Z</DefinedDirection><Source>ReferenceFrame</Source><SourceDirection>+X</SourceDirection><FeatureName></FeatureName></PrimaryAxis><SecondaryAxis><DefinedDirection>+X</DefinedDirection><Source>ReferenceFrame</Source><SourceDirection>+Z</SourceDirection><FeatureName></FeatureName></SecondaryAxis></Value></Frame><Frame><Id>Frame2</Id><Value><Name>one</Name><Origin><Source>GeometricFeature</Source><FeatureName>planar surface 15</FeatureName></Origin><PrimaryAxis><DefinedDirection>+Z</DefinedDirection><Source>ReferenceFrame</Source><SourceDirection>-X</SourceDirection><FeatureName></FeatureName></PrimaryAxis><SecondaryAxis><DefinedDirection>+X</DefinedDirection><Source>ReferenceFrame</Source><SourceDirection>-Z</SourceDirection><FeatureName></FeatureName></SecondaryAxis></Value></Frame><Frame><Id>Frame3</Id><Value><Name>two</Name><Origin><Source>GeometricFeature</Source><FeatureName>planar surface 14</FeatureName></Origin><PrimaryAxis><DefinedDirection>+Z</DefinedDirection><Source>ReferenceFrame</Source><SourceDirection>-X</SourceDirection><FeatureName></FeatureName></PrimaryAxis><SecondaryAxis><DefinedDirection>+X</DefinedDirection><Source>ReferenceFrame</Source><SourceDirection>-Z</SourceDirection><FeatureName></FeatureName></SecondaryAxis></Value></Frame></Frames>
  wall top : sm_lib/Body Elements/File Solid  ExtGeomFileName=Wall Project 2.STEP  UnitType=FromFile  ExtGeomFileUnits=m  StepReaderType=HEX  ExportConvexHullGeometry=off  InertiaType=CalculateFromGeometry  BasedOnType=Mass  Density=1000  DensityUnits=kg/m^3  Mass=1  MassUnits=kg  CenterOfMass=[0 0 0]  CenterOfMassUnits=m  MomentsOfInertia=[1 1 1]  MomentsOfInertiaUnits=kg*m^2  ProductsOfInertia=[0 0 0]  ProductsOfInertiaUnits=kg*m^2  GraphicType=FromGeometry  MarkerShape=Sphere  MarkerSize=10  GraphicVisPropType=SimpleVisualProperties  GraphicDiffuseColor=[0.5 0.5 0.5]  GraphicOpacity=1  GraphicSpecularColor=[0.5 0.5 0.5 1.0]  GraphicAmbientColor=[0.15 0.15 0.15 1.0]  GraphicEmissiveColor=[0.0 0.0 0.0 1.0]  GraphicShininess=75  DoExposeReferenceFrame=off  SerializedFrames=<Frames><Frame><Id>Frame1</Id><Value><Name>F1</Name><Origin><Source>GeometricFeature</Source><FeatureName>circular curve 8</FeatureName></Origin><PrimaryAxis><DefinedDirection>+Z</DefinedDirection><Source>ReferenceFrame</Source><SourceDirection>-X</SourceDirection><FeatureName></FeatureName></PrimaryAxis><SecondaryAxis><DefinedDirection>+X</DefinedDirection><Source>ReferenceFrame</Source><SourceDirection>-Z</SourceDirection><FeatureName></FeatureName></SecondaryAxis></Value></Frame><Frame><Id>Frame2</Id><Value><Name>three</Name><Origin><Source>GeometricFeature</Source><FeatureName>planar surface 14</FeatureName></Origin><PrimaryAxis><DefinedDirection>+Z</DefinedDirection><Source>ReferenceFrame</Source><SourceDirection>+X</SourceDirection><FeatureName></FeatureName></PrimaryAxis><SecondaryAxis><DefinedDirection>+X</DefinedDirection><Source>ReferenceFrame</Source><SourceDirection>+Z</SourceDirection><FeatureName></FeatureName></SecondaryAxis></Value></Frame><Frame><Id>Frame3</Id><Value><Name>four</Name><Origin><Source>GeometricFeature</Source><FeatureName>planar surface 15</FeatureName></Origin><PrimaryAxis><DefinedDirection>+Z</DefinedDirection><Source>ReferenceFrame</Source><SourceDirection>+X</SourceDirection><FeatureName></FeatureName></PrimaryAxis><SecondaryAxis><DefinedDirection>+X</DefinedDirection><Source>ReferenceFrame</Source><SourceDirection>+Z</SourceDirection><FeatureName></FeatureName></SecondaryAxis></Value></Frame></Frames>
  connections:
  free/RConn1 -- forced/RConn1 -- pendulum arm/LConn1
  encoder holder/LConn1 -- peg board/LConn1
  Weld Joint2/RConn1 -- three/LConn1
  one/LConn1 -- pendulum arm/RConn1
  four/LConn2 -- pendulum arm/LConn3
  Mechanism Configuration/RConn1 -- peg board/RConn1 -- World Frame/RConn1 -- Solver Configuration/RConn1
  Rigid Transform4/RConn1 -- Weld Joint3/LConn1
  encoder/RConn1 -- forced/LConn1 -- free/LConn1
  wall top/LConn1 -- peg board/LConn2
  wall bottom/LConn1 -- peg board/RConn2
  Rigid Transform2/LConn1 -- wall bottom/LConn2
  encoder/LConn1 -- encoder holder/RConn1
  Rigid Transform3/RConn1 -- Weld Joint2/LConn1
  Rigid Transform3/LConn1 -- wall top/RConn1
  Rigid Transform4/LConn1 -- wall top/LConn2
  two/LConn2 -- Weld Joint/RConn1
  three/LConn2 -- pendulum arm/RConn2
  four/LConn1 -- Weld Joint3/RConn1
  Weld Joint/LConn1 -- Rigid Transform2/RConn1
  Weld Joint1/LConn1 -- Rigid Transform1/RConn1
  Rigid Transform1/LConn1 -- wall bottom/RConn1
  one/LConn2 -- Weld Joint1/RConn1
  two/LConn1 -- pendulum arm/LConn2
